simulink model "c280x_2833x_adcpwmasynctest_ert"  (R2022b)
settings: Solver=FixedStepDiscrete  StartTime=0.0  StopTime=inf  RelTol=1e-3  EnableMultiTasking=on
undefined symbols (not defined in the file or in its folder): Down, Up
libraries: c280xlib x3, demo_controls x1, c2000lib x1
settings Model: Creator=The MathWorks, Inc.  LastModifiedBy=enzoc
settings SolverCC: AlgebraicLoopSolver=TrustRegion
settings DataIOCC: LimitDataPoints=on  SaveFormat=Array  SaveOutput=off  SaveTime=off  ReturnWorkspaceOutputs=off
settings OptimizationCC: ExpressionDepthLimit=2147483647  InitFltsAndDblsToZero=on  LifeSpan=inf  MaxStackSize=64  EfficientTunableParamExpr=on
settings DebuggingCC: UnderspecifiedInitializationDetection=Classic  MergeDetectMultiDrivingBlocksExec=none  SignalResolutionControl=TryResolveAllWithWarning  InheritedTsInSrcMsg=none  MultiTaskDSMMsg=warning  MultiTaskCondExecSysMsg=none  FcnCallInpInsideContextMsg=warning  UnconnectedInputMsg=warning  UnconnectedOutputMsg=warning  UnconnectedLineMsg=warning  AllowSymbolicDim=off  StateNameClashWarn=warning  SFUnexpectedBacktrackingDiag=warning  SFNoUnconditionalDefaultTransitionDiag=warning  SFExecutionAtInitializationDiag=none  SFMachineParentedDataDiag=warning  ArithmeticOperatorsInVariantConditions=warning
settings HardwareCC: ProdBitPerChar=16  ProdBitPerInt=16  ProdBitPerPointer=32  ProdBitPerSizeT=32  ProdBitPerPtrDiffT=32  ProdLargestAtomicInteger=Integer  ProdLargestAtomicFloat=None  ProdWordSize=16  ProdHWDeviceType=Texas Instruments->C2000  TargetBitPerChar=16  TargetBitPerInt=16  TargetBitPerPointer=16  TargetLargestAtomicInteger=Integer  TargetIntDivRoundTo=Zero  TargetEndianess=LittleEndian  TargetWordSize=16  TargetHWDeviceType=Texas Instruments->C2000  ProdEqTarget=off
settings ModelReferenceCC: EnableRefExpFcnMdlSchedulingChecks=on  PropagateSignalLabelsOutOfModel=off
settings SFSimCC: SimUseLocalCustomCode=off  MATLABDynamicMemAlloc=off  CustomCodeUndefinedFunction=UseInterfaceOnly
settings RTWCC: Description=Embedded Coder  SystemTargetFile=ert.tlc  HardwareBoard=TI Delfino F2833x  TLCOptions=-aInlineSetEventsForThisBaseRateFcn=TLC_FALSE -aSuppressMultiTaskScheduler=TLC_FALSE -aRateBasedStepFcn=1  TemplateMakefile=ert_default_tmf  PostCodeGenCommand=; codertarget.postCodeGenHookCommand(h)  RTWUseLocalCustomCode=off  Toolchain=Texas Instruments Code Composer Studio (C2000)
settings CodeAppCC: IgnoreCustomStorageClasses=off  CustomSymbolStrType=$N$R$M  StateflowObjectComments=on  InternalIdentifier=Classic
settings ERTTargetCC: MultiwordLength=2048  ParMdlRefBuildCompliant=off  CompOptLevelCompliant=off  ConcurrentExecutionCompliant=off  CPPClassGenCompliant=off  ExtModeStaticAllocSize=2048  ExtModeMexFile=TIC2000ExternalModeOpen  ExtModeIntrfLevel=Level2 - Open  ConvertIfToSwitch=off  SuppressUnreachableDefaultCases=off
settings ConfigComp: CovMetricSettings=dw  CovSaveCumulativeToWorkspaceVar=on  CovSaveSingleToWorkspaceVar=on  CovExternalEMLEnable=off  CovSFcnEnable=off

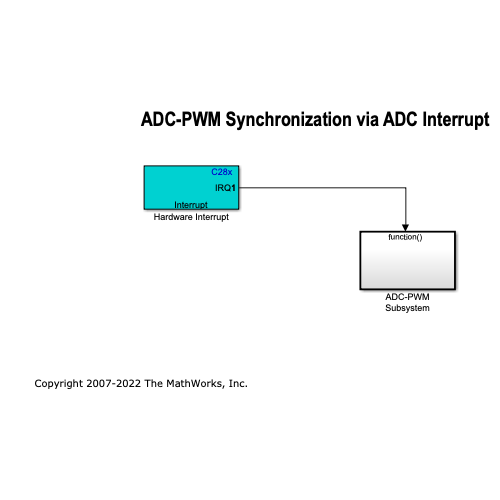
[thumbnail: Simulink's stored preview of the top-level diagram]
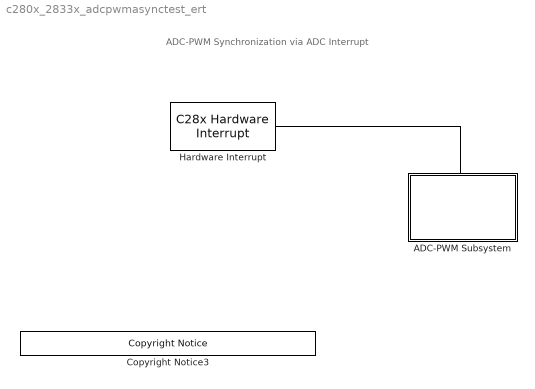
== system c280x_2833x_adcpwmasynctest_ert ==
  note: ADC-PWM Synchronization via ADC Interrupt
  ADC-PWM Subsystem : Subsystem  TreatAsAtomicUnit=on
  Copyright Notice3 : demo_controls/Copyright Notice  year=2007  prod=tic2000
  Hardware Interrupt : c2000lib/Scheduling/C28x Hardware Interrupt  irqnumbers=[1]  pienumbers=[1]  irqpriorities=[30]  irqpreempts=[0]  showinput=off  dspchiptype=C280X
  wires:
  Hardware Interrupt/1 -> ?

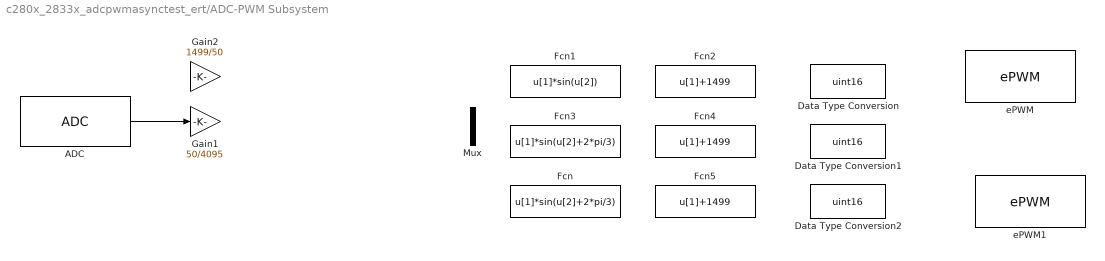
== system c280x_2833x_adcpwmasynctest_ert/ADC-PWM Subsystem ==
  ADC : c280xlib/ADC  useModule=A  useMode=Sequential  sourceSOC=Software  sourceSOC1=ePWMxA  sourceSOC2=ePWMxB  xint2_ADCSOC=31  Ts=-1  dType=uint16  postInterrupt=on  endma=off  chdma=1  numConversionsSingle=1  numConversionsDouble=1  conv0=ADCINA0  conv1=ADCINA1  conv2=ADCINA2  conv3=ADCINA3  conv4=ADCINA4  conv5=ADCINA5  conv6=ADCINA6  conv7=ADCINA7  conv8=ADCINB0  conv9=ADCINB1  conv10=ADCINB2  conv11=ADCINB3  conv12=ADCINB4  conv13=ADCINB5  conv14=ADCINB6  conv15=ADCINB7  convAB0=ADCINA0 and ADCINB0  convAB1=ADCINA1 and ADCINB1  convAB2=ADCINA2 and ADCINB2  convAB3=ADCINA3 and ADCINB3  convAB4=ADCINA4 and ADCINB4  convAB5=ADCINA5 and ADCINB5  convAB6=ADCINA6 and ADCINB6  convAB7=ADCINA7 and ADCINB7  convA0=ADCINA0  convA1=ADCINA1  convA2=ADCINA2  convA3=ADCINA3  convA4=ADCINA4  convA5=ADCINA5  convA6=ADCINA6  convA7=ADCINA7  convB0=ADCINB0  convB1=ADCINB1  convB2=ADCINB2  convB3=ADCINB3  convB4=ADCINB4  convB5=ADCINB5  convB6=ADCINB6  convB7=ADCINB7  c28xmultiPort=off
  Data Type Conversion : DataTypeConversion  OutDataTypeStr=uint16  SaturateOnIntegerOverflow=off  RndMeth=Floor
  Data Type Conversion1 : DataTypeConversion  OutDataTypeStr=uint16  SaturateOnIntegerOverflow=off  RndMeth=Floor
  Data Type Conversion2 : DataTypeConversion  OutDataTypeStr=uint16  SaturateOnIntegerOverflow=off  RndMeth=Floor
  Fcn : Fcn  Expr=u[1]*sin(u[2]+2*pi/3)
  Fcn1 : Fcn  Expr=u[1]*sin(u[2])
  Fcn2 : Fcn  Expr=u[1]+1499
  Fcn3 : Fcn  Expr=u[1]*sin(u[2]+2*pi/3)
  Fcn4 : Fcn  Expr=u[1]+1499
  Fcn5 : Fcn  Expr=u[1]+1499
  Gain1 : Gain  Gain=50/4095  OutDataTypeStr=Inherit: Same as input  ParamDataTypeStr=Inherit: Same as input
  Gain2 : Gain  Gain=1499/50  OutDataTypeStr=Inherit: Same as input  ParamDataTypeStr=Inherit: Same as input
  Mux : Mux  Inputs=2
  ePWM : c280xlib/ePWM  checkMode=off  useModule=ePWM1  periodUnits=Clock cycles  timerSource=Specify via dialog  timerPeriod_clk=2999  timerPeriod_sec=0.0001  tbshadow=Counter equals to zero  countingMode=Up-Down  phaseActiveEnable=Disable  phaseDirection=Count down after sync  phaseActive=0  synchronizationEnable=off  synchronizationOption=Disable  clockPrescale=1  HSclockPrescale=1  ePWMxAStatus=on  CMPAUnits=Clock cycles  CMPASource=Input port  CMPAValue_per=50  CMPAValue_clk=5000  enCMPAshadow=Counter equals to zero  ePWMxAactionLogic1=Set  ePWMxAactionLogic2=Clear  ePWMxAactionLogic3=Clear  ePWMxAactionLogic4=Set  ePWMxAactionLogic5=Do nothing  ePWMxAactionLogic6=Do nothing  ePWMxALoadMode=Freeze  ePWMxACSFenable=off  ePWMxACSFvalue=Forcing disable  ePWMxASFreload=Zero  enHRPWM=off  HRPWM_LoadMode=Counter equals to zero (CTR=ZERO)  HRPWM_CTLMode=Phase control mode  HRPWM_EDGMode=Both edge  enSFO=on  ePWMxBStatus=on  CMPBUnits=Clock cycles  CMPBSource=Specify via dialog  CMPBValue_per=0  CMPBValue_clk=0  enCMPBshadow=Counter equals to zero  ePWMxBactionLogic1=Clear  ePWMxBactionLogic2=Set  ePWMxBactionLogic3=Set  ePWMxBactionLogic4=Clear  ePWMxBactionLogic5=Do nothing  ePWMxBactionLogic6=Do nothing  ePWMxBLoadMode=Load on counter equals to zero (CTR=Zero)  ePWMxBCSFenable=off  ePWMxBCSFvalue=Forcing disable  ePWMxBSFreload=Zero  enableDBePWMxA=on  enableDBePWMxB=on  DBpolarity=Active high complementary (AHC)  DBedgeDelay=Positive  DBSource_ePWMxA=ePWMxA  DBSource_ePWMxB=ePWMxA  DBperiodSource=Specify via dialog  REDperiod=300  FEDperiod=300  adcstartModuleA=on  adcrequestEventA=First event  adcstartEventA=Counter equals to period (CTR=PRD)  adcstartModuleB=off  adcrequestEventB=First event  adcstartEventB=Counter equals to zero (CTR=Zero)  intEn=off  intPrd=First event  intSel=Counter equals to zero (CTR=Zero)  chopperEnable=off  chopperFrequency=1  chopperFirstwidth=1  chopperDuty=12.5%  tripZonesource=Specify via dialog  tzselOSHT1=off  tzselOSHT2=off  tzselOSHT3=off  tzselOSHT4=off  tzselOSHT5=off  tzselOSHT6=off  tzselCBC1=off  tzselCBC2=off  tzselCBC3=off  tzselCBC4=off  tzselCBC5=off  tzselCBC6=off  enTzOstIntr=off  enTzCbcIntr=off  ePWMxAforced=No action  ePWMxBforced=No action  timerPeriod=-1  ePWMxAValue=1  ePWMxBValue=0  tripZoneoption=One-shot trip (OSHT)
  ePWM1 : c280xlib/ePWM  checkMode=off  useModule=ePWM1  periodUnits=Clock cycles  timerSource=Specify via dialog  timerPeriod_clk=2999  timerPeriod_sec=0.0001  tbshadow=Counter equals to zero  countingMode=Up-Down  phaseActiveEnable=Disable  phaseDirection=Count down after sync  phaseActive=0  synchronizationEnable=off  synchronizationOption=Disable  clockPrescale=1  HSclockPrescale=1  ePWMxAStatus=on  CMPAUnits=Clock cycles  CMPASource=Input port  CMPAValue_per=50  CMPAValue_clk=5000  enCMPAshadow=Counter equals to zero  ePWMxAactionLogic1=Set  ePWMxAactionLogic2=Clear  ePWMxAactionLogic3=Clear  ePWMxAactionLogic4=Set  ePWMxAactionLogic5=Do nothing  ePWMxAactionLogic6=Do nothing  ePWMxALoadMode=Freeze  ePWMxACSFenable=off  ePWMxACSFvalue=Forcing disable  ePWMxASFreload=Zero  enHRPWM=off  HRPWM_LoadMode=Counter equals to zero (CTR=ZERO)  HRPWM_CTLMode=Phase control mode  HRPWM_EDGMode=Both edge  enSFO=on  ePWMxBStatus=on  CMPBUnits=Clock cycles  CMPBSource=Specify via dialog  CMPBValue_per=0  CMPBValue_clk=0  enCMPBshadow=Counter equals to zero  ePWMxBactionLogic1=Clear  ePWMxBactionLogic2=Set  ePWMxBactionLogic3=Set  ePWMxBactionLogic4=Clear  ePWMxBactionLogic5=Do nothing  ePWMxBactionLogic6=Do nothing  ePWMxBLoadMode=Load on counter equals to zero (CTR=Zero)  ePWMxBCSFenable=off  ePWMxBCSFvalue=Forcing disable  ePWMxBSFreload=Zero  enableDBePWMxA=on  enableDBePWMxB=on  DBpolarity=Active high complementary (AHC)  DBedgeDelay=Positive  DBSource_ePWMxA=ePWMxA  DBSource_ePWMxB=ePWMxA  DBperiodSource=Specify via dialog  REDperiod=300  FEDperiod=300  adcstartModuleA=on  adcrequestEventA=First event  adcstartEventA=Counter equals to period (CTR=PRD)  adcstartModuleB=off  adcrequestEventB=First event  adcstartEventB=Counter equals to zero (CTR=Zero)  intEn=off  intPrd=First event  intSel=Counter equals to zero (CTR=Zero)  chopperEnable=off  chopperFrequency=1  chopperFirstwidth=1  chopperDuty=12.5%  tripZonesource=Specify via dialog  tzselOSHT1=off  tzselOSHT2=off  tzselOSHT3=off  tzselOSHT4=off  tzselOSHT5=off  tzselOSHT6=off  tzselCBC1=off  tzselCBC2=off  tzselCBC3=off  tzselCBC4=off  tzselCBC5=off  tzselCBC6=off  enTzOstIntr=off  enTzCbcIntr=off  ePWMxAforced=No action  ePWMxBforced=No action  timerPeriod=-1  ePWMxAValue=1  ePWMxBValue=0  tripZoneoption=One-shot trip (OSHT)
  wires:
  ADC/1 -> Gain1/1
